simulink model "ControladorAngularPID"  (R2026b)
settings: Solver=VariableStepAuto
settings Model: Creator=fedeb  LastModifiedBy=fedeb

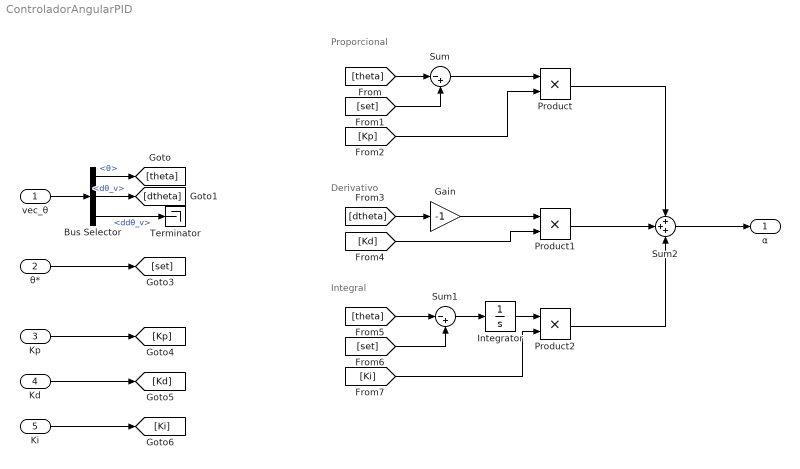
== system ControladorAngularPID ==
  note: Proporcional
  note: Derivativo
  note: Integral
  vec_θ : Inport
  θ* : Inport  Port=2
  Kp : Inport  Port=3
  Kd : Inport  Port=4
  Ki : Inport  Port=5
  Bus Selector : BusSelector  OutputSignals=θ,dθ_v,ddθ_v
  Gain : Gain  Gain=-1
  Integrator : Integrator
  Product : Product
  Product1 : Product
  Product2 : Product
  Sum : Sum  Inputs=|-+
  Sum1 : Sum  Inputs=|-+
  Sum2 : Sum  Inputs=+++
  Terminator : Terminator
  α : Outport
  wires:
  Bus Selector/2 -> [dtheta]  "<dθ_v>"
  Bus Selector/1 -> [theta]  "<θ>"
  vec_θ/1 -> Bus Selector/1
  θ*/1 -> [set]
  [theta] -> Sum/1
  [set] -> Sum/2
  Kp/1 -> [Kp]
  Kd/1 -> [Kd]
  Ki/1 -> [Ki]
  Sum/1 -> Product/1
  [Kp] -> Product/2
  [dtheta] -> Gain/1
  [Kd] -> Product1/2
  Gain/1 -> Product1/1
  [theta] -> Sum1/1
  [set] -> Sum1/2
  [Ki] -> Product2/2
  Sum1/1 -> Integrator/1
  Integrator/1 -> Product2/1
  Product1/1 -> Sum2/2
  Product/1 -> Sum2/1
  Product2/1 -> Sum2/3
  Sum2/1 -> α/1
  Bus Selector/3 -> Terminator/1  "<ddθ_v>"
